simulink model "Path_Planning_Simulink"  (R2025a)
settings: Solver=ode4  StartTime=0.0  StopTime=10.0  FixedStep=.1  RelTol=1e-3
settings Model: Creator=Owner  LastModifiedBy=Owner

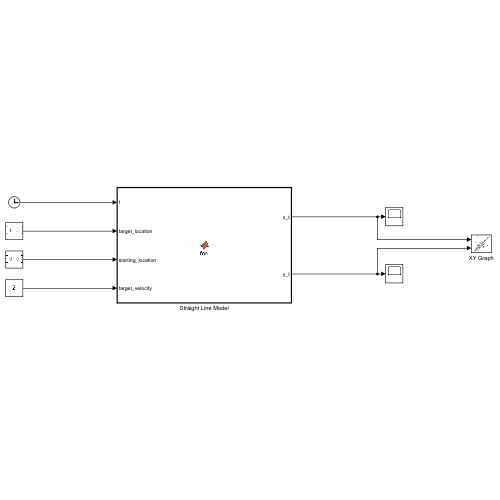
[thumbnail: Simulink's stored preview of the top-level diagram]
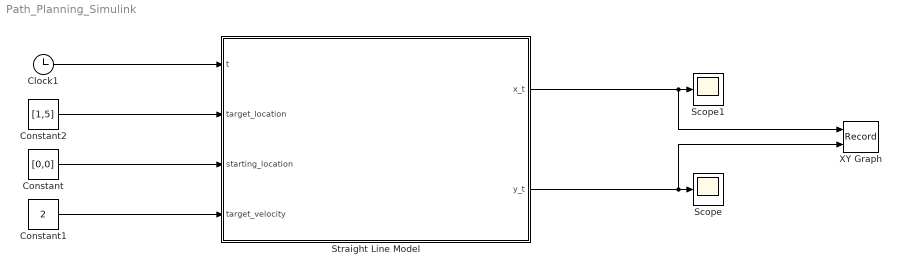
== system Path_Planning_Simulink ==
  Clock1 : Clock
  Constant : Constant  Value=[0,0]  VectorParams1D=off
  Constant1 : Constant  Value=2
  Constant2 : Constant  Value=[1,5]  VectorParams1D=off
  Scope : Scope
      settings: ActiveDisplayYMinimum=-1  ActiveDisplayYMaximum=1
  Scope1 : Scope
      settings: ActiveDisplayYMinimum=-1  ActiveDisplayYMaximum=1
  Straight Line Model : MATLAB Function  TreatAsAtomicUnit=on
  XY Graph : Record  NumPorts=2.0  FileSettingsInternal="{\"entries\":[{\"content\":{\"excelSettings\":{\"content\":{},\"type\":\"Streamout.ExcelSettings\"},\"parquetSettings\":{\"content\":{},\"type\":\"Streamout.ParquetSettings\"}},\"type\":\"Streamout.FileSettingStorage\",\"uuid\":\"\"}],\"packageUris\":[\"http:\\/\\/schema.mathworks.com\\/mf0\\/streamout_blocks\\/R2020a\"],\"version\":\"1.0\"}"  FrameSettings=[0, 0]  Layout=[1 1]  SignalsInternal="{\"entries\":[{\"content\":{\"signals\":[{\"content\":{\"blockPath\":[],\"dimensions\":[1],\"domain\":\"\",\"lineColor\":\"#a2142f\",\"plots\":[ 1 ],\"port\":1,\"sid\":[\"\"],\"signalID\":1,\"signalName\":\"Straight Line Model:1\"},\"type\":\"RecordBlkView.Signal\",\"uuid\":\"\"},{\"content\":{\"blockPath\":[],\"dimensions\":[1],\"domain\":\"\",\"lineColor\":\"#139fff\",\"plots\":[ 1 ],\"port\":2,\"sid\":[\"\"],\"signalID\":2,\"signalName\":\"Straight Line Model:2\"},\"type\":\"RecordBlkView.Signal\",\"uuid\":\"\"}]},\"type\":\"RecordBlkView.InputSignals\",\"uuid\":\"\"}],\"packageUris\":[\"http:\\/\\/schema.mathworks.com\\/mf0\\/streamout_blocks\\/R2020a\"],\"version\":\"1.0\"}"  VisualizationBindings="{\"xyplotplugin\":{\"info\":[{\"series\":[{\"bindingParametersList\":[{\"parameter\":\"X-Axis\",\"signalID\":1,\"signalName\":\"Straight Line Model:1\"},{\"parameter\":\"Y-Axis\",\"signalID\":2,\"signalName\":\"Straight Line Model:2\"}],\"seriesID\":0}],\"subplotID\":1}]}}"  CompatibilityTag=XY
  wires:
  Constant/1 -> Straight Line Model/3(starting_location)
  Clock1/1 -> Straight Line Model/1(t)
  Constant2/1 -> Straight Line Model/2(target_location)
  Constant1/1 -> Straight Line Model/4(target_velocity)
  Straight Line Model/2(y_t) -> XY Graph/2, Scope/1
  Straight Line Model/1(x_t) -> XY Graph/1, Scope1/1

== matlab function Path_Planning_Simulink/Straight Line Model ==
  data: t input; target_location input; starting_location input; target_velocity input; x_t output; y_t output
function [x_t, y_t] = fcn(t, target_location, starting_location, target_velocity)

    distance = norm(target_location - starting_location);
    travel_time = distance / target_velocity;

    if travel_time <= 0
        x_t = target_location(1);
        y_t = target_location(2);
    else
        % Fraction of the trip completed
        fraction = min(t / travel_time, 1);

        % Current position
        x_t = starting_location(1) ...
            + fraction * (target_location(1) - starting_location(1));

        y_t = starting_location(2) ...
            + fraction * (target_location(2) - starting_location(2));
    end
end
